simulink model "Copy_of_W04_D_P"  (R2024b)
settings: Solver=ode4  StartTime=0  StopTime=T_final  FixedStep=h  RelTol=1e-3
values from neighbouring files (symbols this model uses):
  beta_c = 0    [W04_0_setup.m]
  k_neg = cfg.k_neg    [W04_0_setup.m]
  k_pos = cfg.k_pos    [W04_0_setup.m]
  Kp = 300    [W04_0_setup.m]
  mp = 25    [W04_0_setup.m]
  N_max = min(2*y_pont*(T_hi - X_ff/2), 2*y_pont*(X_ff/2 - T_lo))    [W04_0_setup.m]
  port_eff = 1    [W04_0_setup.m]
  psi_step = 10    [W04_0_setup.m]
  rp = [0.05 0 -0.35]'    [W04_0_setup.m]
  t_step = 5    [W04_0_setup.m]
  V_c = 0    [W04_0_setup.m]
  x0 = zeros(12,1)    [W04_0_setup.m]
  X_ff = 60    [W04_0_setup.m]
  y_pont = cfg.y_pont    [W04_0_setup.m]
settings Model: Creator=admin  LastModifiedBy=wkyou
settings DataIOCC: ReturnWorkspaceOutputs=off

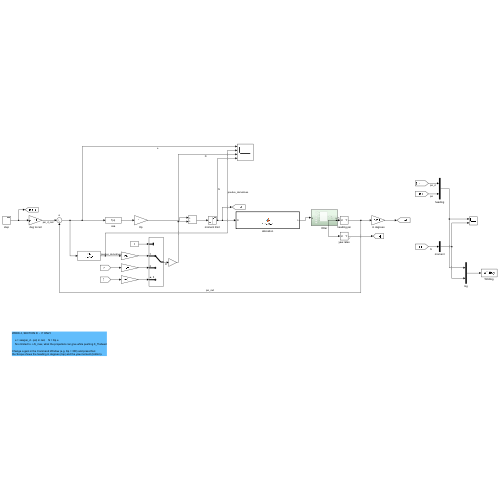
[thumbnail: Simulink's stored preview of the top-level diagram]
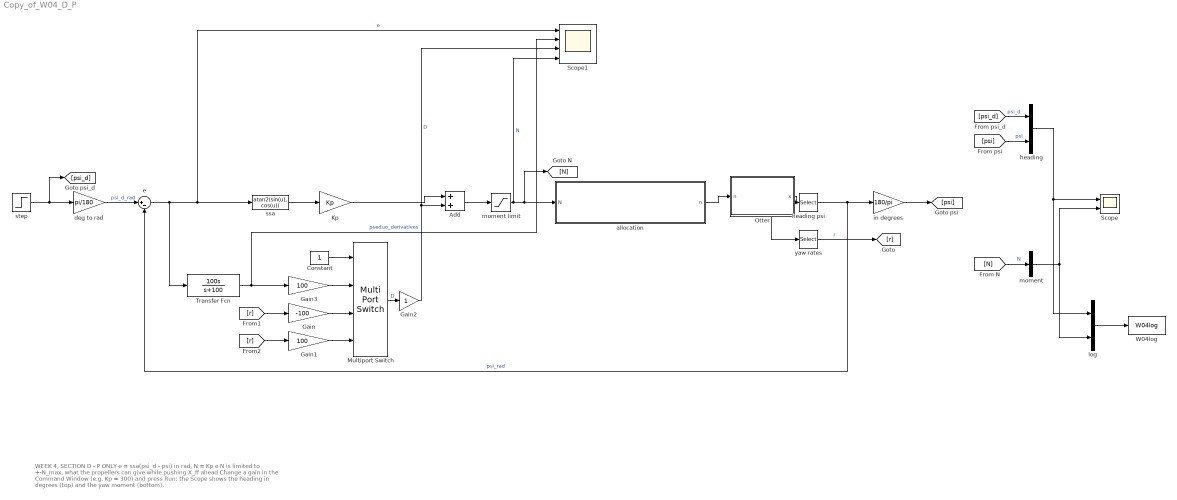
== system Copy_of_W04_D_P ==
  note: WEEK 4, SECTION D  -  P ONLY
      |
      |     e = ssa(psi_d - psi) in rad,    N = Kp e
      |     N is limited to +-N_max, what the propellers can give while pushing X_ff ahead
      |
      | Change a gain in the Command Window (e.g. Kp = 300) and press Run:
      | the Scope shows the heading in degrees (top) and the yaw moment (bottom).
  Add : Sum
  Constant : Constant
  Gain : Gain  Gain=-100
  Gain1 : Gain  Gain=100
  Gain2 : Gain
  Gain3 : Gain  Gain=100
  Kp : Gain  Gain=Kp
  Multiport Switch : MultiPortSwitch  SaturateOnIntegerOverflow=off  InputSameDT=off
  Otter : Subsystem
  Scope : Scope  NumInputPorts=2
  Scope1 : Scope  NumInputPorts=4
  Transfer Fcn : TransferFcn  Numerator=[100 0]  Denominator=[1 100]
  W04log : ToWorkspace  VariableName=W04log  SaveFormat=Structure With Time  SampleTime=-1
  allocation : MATLAB Function  TreatAsAtomicUnit=on
  deg to rad : Gain  Gain=pi/180
  e : Sum  Inputs=|+-
  heading : Mux  Inputs=2
  heading psi : Selector  InputPortWidth=12  IndexOptions=Index vector (dialog)  Indices=12  OutputSizes=1
  in degrees : Gain  Gain=180/pi
  log : Mux  Inputs=2
  moment : Mux  Inputs=1
  moment limit : Saturate  UpperLimit=N_max  LowerLimit=-N_max
  ssa : Fcn  Expr=atan2(sin(u), cos(u))
  step : Step  Time=t_step  After=psi_step  SampleTime=0
  yaw rates : Selector  InputPortWidth=12  IndexOptions=Index vector (dialog)  Indices=6  OutputSizes=1
  wires:
  step/1 -> [psi_d], deg to rad/1
  deg to rad/1 -> e/1  "psi_d_rad"
  e/1 -> Scope1/1, ssa/1, Transfer Fcn/1  "e"
  ssa/1 -> Kp/1
  Add/1 -> moment limit/1
  moment limit/1 -> Scope1/4, [N], allocation/1(N)  "N"
  allocation/1(n) -> Otter/1(n)
  Otter/1(x) -> yaw rates/1, heading psi/1
  heading psi/1 -> e/2, in degrees/1  "psi_rad"
  in degrees/1 -> [psi]
  [psi_d] -> heading/1  "psi_d"
  [psi] -> heading/2  "psi"
  [N] -> moment/1  "N"
  heading/1 -> Scope/1, log/1
  moment/1 -> Scope/2, log/2
  log/1 -> W04log/1
  Kp/1 -> Add/1
  Gain2/1 -> Scope1/3, Add/2  "D"
  Constant/1 -> Multiport Switch/1
  Transfer Fcn/1 -> Gain3/1, Scope1/2  "pseduo_derivatives"
  yaw rates/1 -> [r]  "r"
  Gain/1 -> Multiport Switch/3
  [r] -> Gain/1
  [r] -> Gain1/1
  Gain1/1 -> Multiport Switch/4
  Multiport Switch/1 -> Gain2/1  "D"
  Gain3/1 -> Multiport Switch/2

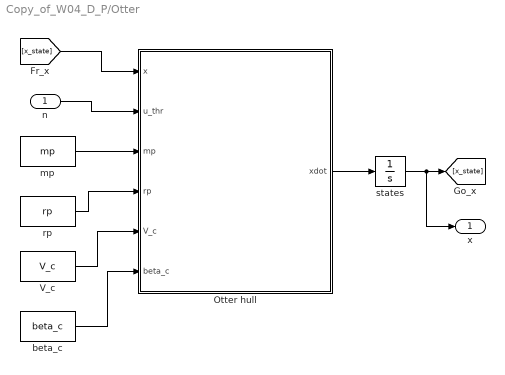
== system Copy_of_W04_D_P/Otter ==
  n : Inport
  Otter hull : MATLAB Function  TreatAsAtomicUnit=on
  V_c : Constant  Value=V_c
  beta_c : Constant  Value=beta_c
  mp : Constant  Value=mp
  rp : Constant  Value=rp
  states : Integrator  InitialCondition=x0
  x : Outport
  wires:
  [x_state] -> Otter hull/1(x)
  rp/1 -> Otter hull/4(rp)
  n/1 -> Otter hull/2(u_thr)
  states/1 -> [x_state], x/1
  V_c/1 -> Otter hull/5(V_c)
  mp/1 -> Otter hull/3(mp)
  beta_c/1 -> Otter hull/6(beta_c)
  Otter hull/1(xdot) -> states/1

== matlab function Copy_of_W04_D_P/Otter/Otter hull ==
  data: x input; xdot output double size=[12 1]; u_thr input; mp input; rp input; V_c input; beta_c input
function xdot = otter_hull(x, u_thr, mp, rp, V_c, beta_c)
% Fossen's otter.m, called unchanged from Tools/MSS/VESSELS.
%
%   x       12 states, fed back from the integrator
%   u_thr   propeller shaft speeds [rad/s]
%
% otter.m is not written for code generation, so the call is extrinsic and
% xdot has to be pre-sized for Simulink to know the output width.
coder.extrinsic('otter');

xdot = zeros(12,1);
xdot = otter(x, u_thr, mp, rp, V_c, beta_c);
end

== matlab function Copy_of_W04_D_P/allocation ==
  data: N input; n output double size=[2 1]; X_ff parameter; y_pont parameter; k_pos parameter; k_neg parameter; port_eff parameter
function n = allocation(N, X_ff, y_pont, k_pos, k_neg, port_eff)
%#codegen
%ALLOCATION  요 모멘트 N [N m] 를 두 프로펠러의 축 회전수 n [rad/s] 로 바꾼다.
%            Turn the yaw moment N [N m] into the shaft speeds n [rad/s] of the two propellers.
%
%   N 만 입력 포트다. 나머지는 작업공간 변수 (W04_0_setup) 에서 온다.
%   Only N is an input port; the rest come from the workspace (W04_0_setup).
%     X_ff      두 프로펠러가 함께 내는 전진력 / surge force from both propellers   [N]
%     y_pont    중심선에서 각 프로펠러까지의 거리 / each propeller's arm              [m]
%     k_pos     앞으로 밀 때 추력 계수 / thrust coefficient ahead
%     k_neg     뒤로 당길 때 추력 계수 / thrust coefficient astern
%     port_eff  좌현 프로펠러 효율, 보통 1 (절 F 는 0.7) / port efficiency, 1 unless section F

% 1) 두 프로펠러의 추력. 둘 다 X_ff 의 절반씩 밀고, 모멘트는 한쪽을 더 세게,
%    다른 쪽을 덜 세게 밀어 만든다. 팔 길이가 y_pont 이므로
%        y_pont (T1 - T2) = N,   T1 + T2 = X_ff
%    Both push half of X_ff ahead; the moment comes from pushing one side
%    harder and the other less. With arm y_pont:
%        y_pont (T1 - T2) = N,   T1 + T2 = X_ff
T = [X_ff/2 + N/(2*y_pont);      % 좌현 / port
     X_ff/2 - N/(2*y_pont)];     % 우현 / starboard

% 2) 약한 좌현 프로펠러: 요구한 추력의 port_eff 배만 낸다 (절 F).
%    A weak port propeller delivers only port_eff of what is asked (section F).
T(1) = port_eff * T(1);

% 3) 프로펠러 곡선 T = k n|n| (1주차) 을 하나씩 n 에 대해 푼다.
%    앞으로와 뒤로의 계수가 다르다 (k_pos > k_neg).
%    Solve the propeller curve T = k n|n| (Week 1) for each n; the coefficient
%    differs ahead and astern (k_pos > k_neg).
n = zeros(2,1);
for i = 1:2
    if T(i) >= 0
        n(i) =  sqrt( T(i) / k_pos);   % 앞으로 / ahead
    else
        n(i) = -sqrt(-T(i) / k_neg);   % 뒤로 / astern
    end
end
end
